simulink subsystem "Vehicle1D_Custom_refsub"  (R2025a)
settings: Solver=VariableStepAuto  StartTime=0.0  StopTime=10.0  RelTol=1e-3
libraries: nesl_utility x6, fl_lib x2
settings Model: Creator=isaacito  LastModifiedBy=isaacito
settings SolverCC: AlgebraicLoopSolver=TrustRegion
settings DebuggingCC: UnconnectedInputMsg=warning  UnconnectedOutputMsg=warning  UnconnectedLineMsg=warning
settings ModelReferenceCC: EnableRefExpFcnMdlSchedulingChecks=on
settings RTWCC: GPUComputeCapability=3.5  DLArmComputeVersion=19.05

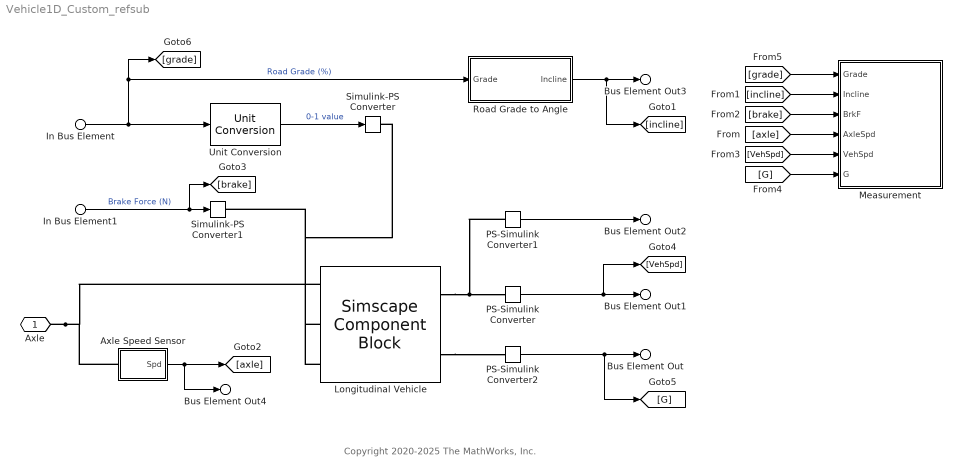
== system Vehicle1D_Custom_refsub ==
  note: Copyright 2020-2025 The MathWorks, Inc.
  In Bus Element : Inport  PortName=Inputs  Element=RoadGrade
      settings: AttributesFormatString=%<Unit>
  In Bus Element1 : Inport  PortName=Inputs  Element=BrakeForce
      settings: AttributesFormatString=%<Unit>
  Axle Speed Sensor : Subsystem
  Longitudinal Vehicle : SimscapeComponentBlock  SourceFile=Vehicle1D_Custom  ComponentPath=Vehicle1D_Custom  ComponentVariants="[\"Vehicle1D_Custom\"]"  ComponentVariantNames="[\"Vehicle1D_Custom\"]"  ClassName=Vehicle1D_Custom  SchemaVersion=1  grav=vehicle.roadLoad_gravAccel_m_per_s2 m/s^2  M_e=vehicle.mass_kg kg  R_tire=vehicle.tireRollingRadius_m m  A_rl=vehicle.roadLoadA_N N  B_rl=vehicle.roadLoadB_N_per_kph N*hr/km  C_rl=vehicle.roadLoadC_N_per_kph2 N*hr^2/km^2  V_1=smoothing.vehicle_speedThreshold_kph km/hr  w_1=smoothing.vehicle_axleSpeedThreshold_rpm rpm  V_x_specify=on  V_x_priority=High  V_x=initial.vehicle_speed_kph km/hr  V_x_nominal_specify=off  V_x_nominal_value=1  V_x_nominal_unit=km/hr
      settings: AttributesFormatString=%<V_x>  CopyFcn=simscape.sscblock.internal.componentBlockCallback(gcbh,'COPY')  PreCopyFcn=simscape.sscblock.internal.componentBlockCallback(gcbh,'PRECOPY')  PreDeleteFcn=simscape.sscblock.internal.componentBlockCallback(gcbh,'PREDELETE')  LogSimulationData=on  InternalSimscapePortConfiguration="{\"Bottom\":[],\"Left\":[{\"id\":\"Axle\",\"label\":\"Axle\",\"type\":\"foundation.mechanical.rotational.rotational\"}],\"Right\":[{\"id\":\"v_out\",\"label\":\"V\",\"type\":\"output\"},{\"id\":\"G\",\"label\":\"G\",\"type\":\"output\"}],\"Top\":[{\"id\":\"brkF\",\"label\":\"Brake\",\"type\":\"input\"},{\"id\":\"grade_norm\",\"label\":\"Grade\",\"type\":\"input\"}]}"
      mask Type: Custom Longitudinal Vehicle
  Measurement : Subsystem
  PS-Simulink Converter : nesl_utility/PS-Simulink Converter  PhysicalDomain=network_engine_domain  SubClassName=ps_output  LeftPortType=input  RightPortType=output  PseudoPeriodic=off  Frequencies=[]  VectorFormat=1-D array  Unit=km/hr  AffineConversion=off
  PS-Simulink Converter1 : nesl_utility/PS-Simulink Converter  PhysicalDomain=network_engine_domain  SubClassName=ps_output  LeftPortType=input  RightPortType=output  PseudoPeriodic=off  Frequencies=[]  VectorFormat=1-D array  Unit=mph  AffineConversion=off
  PS-Simulink Converter2 : nesl_utility/PS-Simulink Converter  PhysicalDomain=network_engine_domain  SubClassName=ps_output  LeftPortType=input  RightPortType=output  PseudoPeriodic=off  Frequencies=[]  VectorFormat=1-D array  Unit=1  AffineConversion=off
  Road Grade to Angle : Subsystem
  Simulink-PS Converter : nesl_utility/Simulink-PS Converter  PhysicalDomain=network_engine_domain  SubClassName=ps_input  LeftPortType=input  RightPortType=output  PseudoPeriodic=off  Frequencies=[]  NoiseDistribution=none  NoiseParameters=[]  Unit=1  AffineConversion=off  FilteringAndDerivatives=filter  SimscapeFilterOrder=1  InputFilterTimeConstant=0.001  UdotUserProvided=0
  Simulink-PS Converter1 : nesl_utility/Simulink-PS Converter  PhysicalDomain=network_engine_domain  SubClassName=ps_input  LeftPortType=input  RightPortType=output  PseudoPeriodic=off  Frequencies=[]  NoiseDistribution=none  NoiseParameters=[]  Unit=N  AffineConversion=off  FilteringAndDerivatives=filter  SimscapeFilterOrder=1  InputFilterTimeConstant=0.001  UdotUserProvided=0
  Unit Conversion : UnitConversion  OutputType=Inherit: Inherit via back propagation
  Axle : PMIOPort  Side=Left
  Bus Element Out : Outport  PortName=Info  Element=G
      settings: AttributesFormatString=%<Unit>
  Bus Element Out1 : Outport  PortName=Info  Element=VehSpdKph
      settings: AttributesFormatString=%<Unit>
  Bus Element Out2 : Outport  PortName=Info  Element=VehSpdMph
      settings: AttributesFormatString=%<Unit>
  Bus Element Out3 : Outport  PortName=Info  Element=Incline
      settings: AttributesFormatString=%<Unit>
  Bus Element Out4 : Outport  PortName=Info  Element=AxleSpd
      settings: AttributesFormatString=%<Unit>
  wires:
  PS-Simulink Converter/1 -> [VehSpd], Bus Element Out1/1
  PS-Simulink Converter2/1 -> [G], Bus Element Out/1
  In Bus Element/1 -> Unit Conversion/1, [grade], Road Grade to Angle/1(Grade)  "Road Grade (%)"
  In Bus Element1/1 -> [brake], Simulink-PS Converter1/1  "Brake Force (N)"
  Unit Conversion/1 -> Simulink-PS Converter/1  "0-1 value"
  PS-Simulink Converter1/1 -> Bus Element Out2/1
  Road Grade to Angle/1(Incline) -> Bus Element Out3/1, [incline]
  Axle Speed Sensor/1(Spd) -> [axle], Bus Element Out4/1
  [incline] -> Measurement/2(Incline)
  [brake] -> Measurement/3(BrkF)
  [axle] -> Measurement/4(AxleSpd)
  [VehSpd] -> Measurement/5(VehSpd)
  [G] -> Measurement/6(G)
  [grade] -> Measurement/1(Grade)
  connections:
  Longitudinal Vehicle/RConn1 -- PS-Simulink Converter/LConn1 -- PS-Simulink Converter1/LConn1
  Axle/RConn1 -- Axle Speed Sensor/LConn1 -- Longitudinal Vehicle/LConn1
  Longitudinal Vehicle/RConn2 -- PS-Simulink Converter2/LConn1
  Longitudinal Vehicle/LConn3 -- Simulink-PS Converter/RConn1
  Longitudinal Vehicle/LConn2 -- Simulink-PS Converter1/RConn1

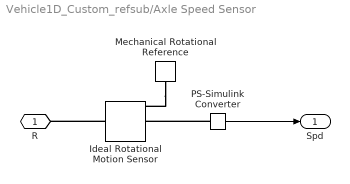
== system Vehicle1D_Custom_refsub/Axle Speed Sensor ==
  Ideal Rotational Motion Sensor : fl_lib/Mechanical/Mechanical Sensors/Ideal Rotational Motion Sensor  reference=foundation.enum.MeasurementReference.difference  acceleration_port=false  velocity_port=true  position_port=true  wrap_angle=simscape.enum.onoff.off  offset=0 rad
  Mechanical Rotational Reference : fl_lib/Mechanical/Rotational Elements/Mechanical Rotational Reference
  PS-Simulink Converter : nesl_utility/PS-Simulink Converter  PhysicalDomain=network_engine_domain  SubClassName=ps_output  LeftPortType=input  RightPortType=output  PseudoPeriodic=off  Frequencies=[]  VectorFormat=1-D array  Unit=rpm  AffineConversion=off
  R : PMIOPort  Side=Left
  Spd : Outport  Unit=rpm
  wires:
  PS-Simulink Converter/1 -> Spd/1
  connections:
  Mechanical Rotational Reference/LConn1 -- Ideal Rotational Motion Sensor/RConn1
  PS-Simulink Converter/LConn1 -- Ideal Rotational Motion Sensor/RConn2
  Ideal Rotational Motion Sensor/LConn1 -- R/RConn1

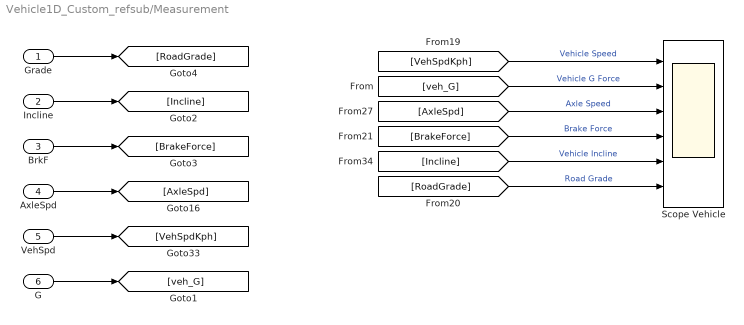
== system Vehicle1D_Custom_refsub/Measurement ==
  Grade : Inport
  Incline : Inport  Port=2
  BrkF : Inport  Port=3
  AxleSpd : Inport  Port=4
  VehSpd : Inport  Port=5
  G : Inport  Port=6
  Scope Vehicle : Scope  NumInputPorts=6
      settings: ActiveDisplayYMinimum=-12.00926  ActiveDisplayYMaximum=102.7511
  wires:
  [VehSpdKph] -> Scope Vehicle/1  "Vehicle Speed"
  [veh_G] -> Scope Vehicle/2  "Vehicle G Force"
  AxleSpd/1 -> [AxleSpd]
  VehSpd/1 -> [VehSpdKph]
  G/1 -> [veh_G]
  Incline/1 -> [Incline]
  BrkF/1 -> [BrakeForce]
  [AxleSpd] -> Scope Vehicle/3  "Axle Speed"
  [BrakeForce] -> Scope Vehicle/4  "Brake Force"
  [Incline] -> Scope Vehicle/5  "Vehicle Incline"
  [RoadGrade] -> Scope Vehicle/6  "Road Grade"
  Grade/1 -> [RoadGrade]

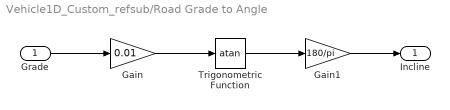
== system Vehicle1D_Custom_refsub/Road Grade to Angle ==
  Grade : Inport  Unit=%
      settings: AttributesFormatString=%<Unit>
  Gain : Gain  Gain=0.01
  Gain1 : Gain  Gain=180/pi
  Trigonometric Function : Trigonometry  Operator=atan
  Incline : Outport  Unit=deg
      settings: AttributesFormatString=%<Unit>
  wires:
  Gain1/1 -> Incline/1
  Trigonometric Function/1 -> Gain1/1
  Grade/1 -> Gain/1
  Gain/1 -> Trigonometric Function/1
